simulink model "modele_codeur_registre"  (R2024b)
settings: Solver=FixedStepDiscrete  StartTime=0.0  StopTime=7*Nw*Tc  FixedStep=Tc  RelTol=1e-3
undefined symbols (not defined in the file or in its folder): Tc
settings Model: Creator=youka  LastModifiedBy=youka

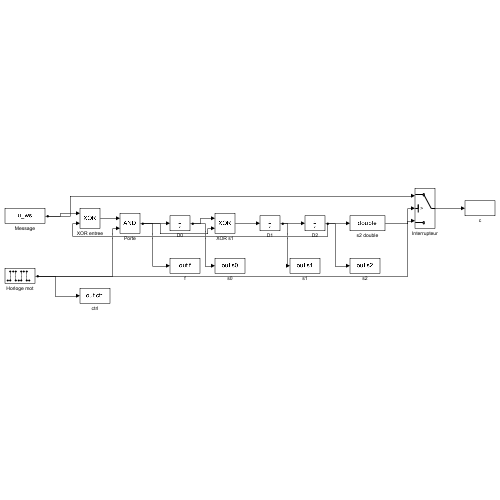
[thumbnail: Simulink's stored preview of the top-level diagram]
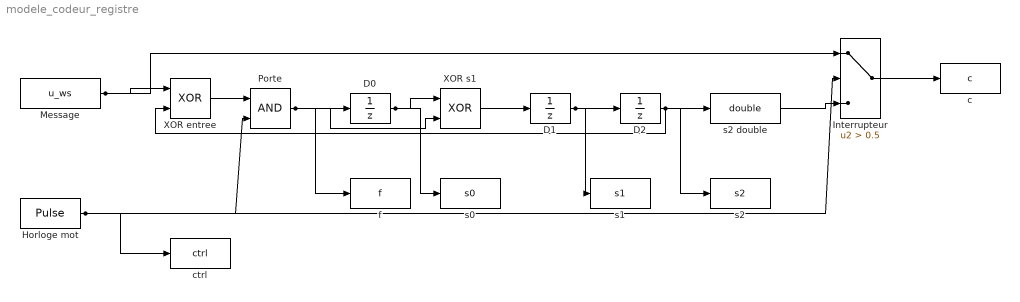
== system modele_codeur_registre ==
  D0 : UnitDelay  SampleTime=Tc  HasFrameUpgradeWarning=on
  D1 : UnitDelay  SampleTime=Tc  HasFrameUpgradeWarning=on
  D2 : UnitDelay  SampleTime=Tc  HasFrameUpgradeWarning=on
  Horloge mot : DiscretePulseGenerator  Period=7  PulseWidth=4  SampleTime=Tc
  Interrupteur : Switch  Criteria=u2 > Threshold  Threshold=0.5  SaturateOnIntegerOverflow=off  InputSameDT=off
  Message : FromWorkspace  VariableName=u_ws  SampleTime=Tc  Interpolate=off  OutputAfterFinalValue=Setting to zero
  Porte : Logic  AllPortsSameDT=off  OutDataTypeStr=boolean
  XOR entree : Logic  Operator=XOR  AllPortsSameDT=off  OutDataTypeStr=boolean
  XOR s1 : Logic  Operator=XOR  AllPortsSameDT=off  OutDataTypeStr=boolean
  c : ToWorkspace  VariableName=c  SampleTime=-1
  ctrl : ToWorkspace  VariableName=ctrl  SampleTime=-1
  f : ToWorkspace  VariableName=f  SampleTime=-1
  s0 : ToWorkspace  VariableName=s0  SampleTime=-1
  s1 : ToWorkspace  VariableName=s1  SampleTime=-1
  s2 : ToWorkspace  VariableName=s2  SampleTime=-1
  s2 double : DataTypeConversion  OutDataTypeStr=double  SaturateOnIntegerOverflow=off  RndMeth=Floor
  wires:
  Message/1 -> XOR entree/1, Interrupteur/1
  D2/1 -> XOR entree/2, s2 double/1, s2/1
  XOR entree/1 -> Porte/1
  Horloge mot/1 -> Porte/2, Interrupteur/2, ctrl/1
  Porte/1 -> D0/1, XOR s1/2, f/1
  D0/1 -> XOR s1/1, s0/1
  XOR s1/1 -> D1/1
  D1/1 -> D2/1, s1/1
  s2 double/1 -> Interrupteur/3
  Interrupteur/1 -> c/1
